simulink model "StampFly_KF400"  (R2026b)
settings: Solver=FixedStepDiscrete  StopTime=inf  FixedStep=Official.Step
PostLoadFcn:
  | run(fullfile(fileparts(get_param('StampFly_KF400','FileName')),'config','startup.m'));
InitFcn:
  | init_kf_flight;
undefined symbols (not defined in the file): AltitudeKF, Bottom, Discrete, Official, Time
libraries: slpidlib x7, simulink x4, ctrlSharedLib x1, mspfiltlib x1
(part 2 of 4)

== system StampFly_KF400/BottomRangeSensor400/BottomToF400 ==
  FinalMode : Inport
  BottomRangeBus : BusCreator  Inputs=2
  PreviousMode : UnitDelay  InitialCondition=uint8(0)  SampleTime=Official.Step
  RangeDiagnosticsBus : BusCreator  Inputs=3
  ToFReadyPoll400 : MATLABSystem  Description=下向きToF：Medium、33 ms。起動時のStartMeasurementは1回。dcnt>14とready割り込みでcore0へ読み出しを要求し、400 Hz側は待たず最新結果を取得。状態0の最遠対象[mm]、新着フラグ、測定状態を出力。前向きToFはXSHUT=LOWで無効。  Priority=3  System=official.BottomToF400  Sensor=Bottom (0x29)  I2CAddress=uint8( 41 )  SampleTime=Official.Step  DistanceMode=Auto (bottom Medium / front Long)  TimingBudget=20  PerformBringUp=on  TargetSelect=Auto (bottom Farthest / front Nearest)  SimulateUsing=Code generation
      mask Type: official.BottomToF400
  BottomRange : Outport
  RangeDiagnostics : Outport  Port=2
  wires:
  BottomRangeBus/1 -> BottomRange/1  "BottomRange"
  ToFReadyPoll400/5 -> RangeDiagnosticsBus/3  "Info"
  ToFReadyPoll400/4 -> RangeDiagnosticsBus/2  "Status"
  ToFReadyPoll400/3 -> RangeDiagnosticsBus/1  "FrontDistanceMm"
  FinalMode/1 -> PreviousMode/1
  ToFReadyPoll400/2 -> BottomRangeBus/2  "Fresh"
  PreviousMode/1 -> ToFReadyPoll400/1
  ToFReadyPoll400/1 -> BottomRangeBus/1  "DistanceMm"
  RangeDiagnosticsBus/1 -> RangeDiagnostics/1  "RangeDiagnostics"

== system StampFly_KF400/BottomRangeSensor400/JapaneseExplanation ==

== system StampFly_KF400/CommandPreparation400/FlightInputBus400 ==
  JoystickCommand : Inport
  BatteryVoltage : Inport  Port=2
  Dt : Inport  Port=3
  SensorStatus : Inport  Port=4
  CommandTapBus : BusCreator  Inputs=2
  ControlInputs : BusCreator  Inputs=7
  JoystickCommandFields : BusSelector  OutputSignals=Sticks,ArmButton,NewPacket,AHRSRequest
  SensorStatusFields : BusSelector  OutputSignals=Flags,Diagnostics
  SensorTapBus : BusCreator  Inputs=2
  FlightInputs : Outport
  CommandTap : Outport  Port=2
  SensorTap : Outport  Port=3
  wires:
  CommandTapBus/1 -> CommandTap/1  "CommandTap"
  SensorStatusFields/1 -> SensorTapBus/1, ControlInputs/7  "<Flags>"
  Dt/1 -> ControlInputs/6
  BatteryVoltage/1 -> ControlInputs/5
  JoystickCommandFields/4 -> CommandTapBus/2, ControlInputs/4  "<AHRSRequest>"
  ControlInputs/1 -> FlightInputs/1  "FlightInputs"
  JoystickCommand/1 -> JoystickCommandFields/1
  JoystickCommandFields/3 -> ControlInputs/3  "<NewPacket>"
  JoystickCommandFields/2 -> ControlInputs/2  "<ArmButton>"
  SensorStatus/1 -> SensorStatusFields/1
  JoystickCommandFields/1 -> CommandTapBus/1, ControlInputs/1  "<Sticks>"
  SensorStatusFields/2 -> SensorTapBus/2  "<Diagnostics>"
  SensorTapBus/1 -> SensorTap/1  "SensorTap"

== system StampFly_KF400/CommandPreparation400/JapaneseExplanation ==

== system StampFly_KF400/DataLogging50/JapaneseExplanation ==

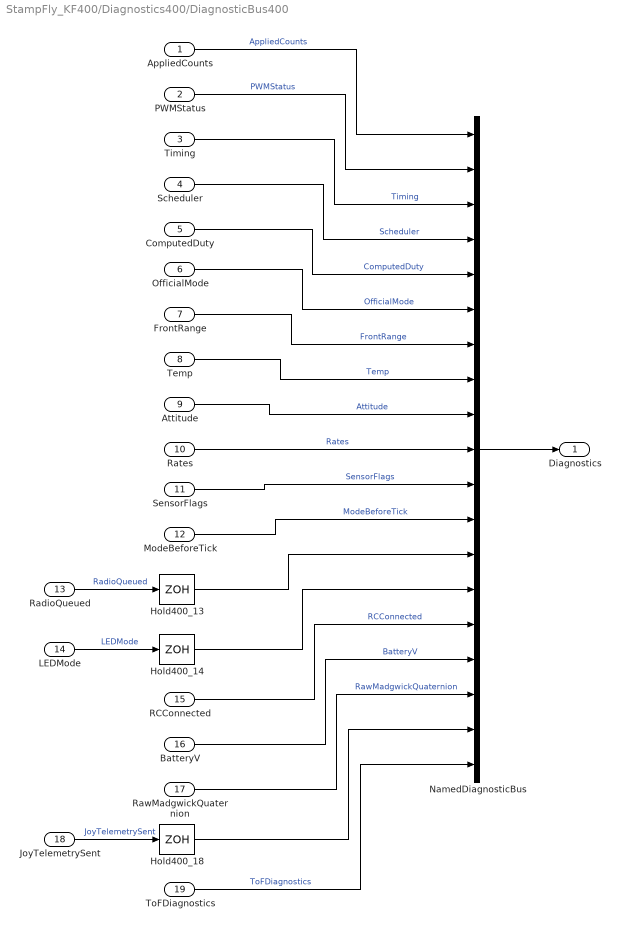
== system StampFly_KF400/Diagnostics400/DiagnosticBus400 ==
  AppliedCounts : Inport
  PWMStatus : Inport  Port=2
  Timing : Inport  Port=3
  Scheduler : Inport  Port=4
  ComputedDuty : Inport  Port=5
  OfficialMode : Inport  Port=6
  FrontRange : Inport  Port=7
  Temp : Inport  Port=8
  Attitude : Inport  Port=9
  Rates : Inport  Port=10
  SensorFlags : Inport  Port=11
  ModeBeforeTick : Inport  Port=12
  RadioQueued : Inport  Port=13
  LEDMode : Inport  Port=14
  RCConnected : Inport  Port=15
  BatteryV : Inport  Port=16
  RawMadgwickQuaternion : Inport  Port=17
  JoyTelemetrySent : Inport  Port=18
  ToFDiagnostics : Inport  Port=19
  Hold400_13 : ZeroOrderHold  SampleTime=.0025
  Hold400_14 : ZeroOrderHold  SampleTime=.0025
  Hold400_18 : ZeroOrderHold  SampleTime=.0025
  NamedDiagnosticBus : BusCreator  Inputs=19  OutDataTypeStr=Bus: OfficialDiagnosticBus  NonVirtualBus=on
  Diagnostics : Outport
  wires:
  RadioQueued/1 -> Hold400_13/1  "RadioQueued"
  ComputedDuty/1 -> NamedDiagnosticBus/5  "ComputedDuty"
  ModeBeforeTick/1 -> NamedDiagnosticBus/12  "ModeBeforeTick"
  Scheduler/1 -> NamedDiagnosticBus/4  "Scheduler"
  ToFDiagnostics/1 -> NamedDiagnosticBus/19  "ToFDiagnostics"
  SensorFlags/1 -> NamedDiagnosticBus/11  "SensorFlags"
  Timing/1 -> NamedDiagnosticBus/3  "Timing"
  Rates/1 -> NamedDiagnosticBus/10  "Rates"
  JoyTelemetrySent/1 -> Hold400_18/1  "JoyTelemetrySent"
  PWMStatus/1 -> NamedDiagnosticBus/2  "PWMStatus"
  RawMadgwickQuaternion/1 -> NamedDiagnosticBus/17  "RawMadgwickQuaternion"
  Attitude/1 -> NamedDiagnosticBus/9  "Attitude"
  AppliedCounts/1 -> NamedDiagnosticBus/1  "AppliedCounts"
  Hold400_14/1 -> NamedDiagnosticBus/14
  OfficialMode/1 -> NamedDiagnosticBus/6  "OfficialMode"
  LEDMode/1 -> Hold400_14/1  "LEDMode"
  RCConnected/1 -> NamedDiagnosticBus/15  "RCConnected"
  FrontRange/1 -> NamedDiagnosticBus/7  "FrontRange"
  BatteryV/1 -> NamedDiagnosticBus/16  "BatteryV"
  Temp/1 -> NamedDiagnosticBus/8  "Temp"
  Hold400_13/1 -> NamedDiagnosticBus/13
  Hold400_18/1 -> NamedDiagnosticBus/18
  NamedDiagnosticBus/1 -> Diagnostics/1

== system StampFly_KF400/EstimatorContext400/JapaneseExplanation ==

== system StampFly_KF400/FlightControl400/JapaneseExplanation ==

== system StampFly_KF400/FlightControl400/PreviousCycle400 ==
  ControlState : Inport
  SupervisorReset : Inport  Port=2
  AHRSResetMemory : UnitDelay  InitialCondition=false  SampleTime=Official.Step
  AltFlagMemory : UnitDelay  InitialCondition=uint8(0)  SampleTime=Official.Step
  AltFlagUInt8 : DataTypeConversion  OutDataTypeStr=uint8  SaturateOnIntegerOverflow=off  RndMeth=Floor
  ControlStateFields : BusSelector  OutputSignals=AltitudeEnabled,Mode
  EstimatorFeedbackBus : BusCreator  Inputs=4
  ModeMemory : UnitDelay  InitialCondition=uint8(0)  SampleTime=Official.Step
  ParkingResetMemory : UnitDelay  InitialCondition=false  SampleTime=Official.Step
  SupervisorResetFields : BusSelector  OutputSignals=AttitudeReset,ParkingReset
  EstimatorFeedback : Outport
  PreviousMode : Outport  Port=2
  AltitudeEnabled : Outport  Port=3
  wires:
  ControlStateFields/1 -> AltFlagUInt8/1  "<AltitudeEnabled>"
  SupervisorResetFields/1 -> AHRSResetMemory/1  "<AttitudeReset>"
  AltFlagMemory/1 -> EstimatorFeedbackBus/2  "AltitudeEnabled"
  ModeMemory/1 -> EstimatorFeedbackBus/1, PreviousMode/1  "PreviousMode"
  SupervisorReset/1 -> SupervisorResetFields/1
  ControlState/1 -> ControlStateFields/1
  ControlStateFields/2 -> ModeMemory/1  "<Mode>"
  SupervisorResetFields/2 -> ParkingResetMemory/1  "<ParkingReset>"
  ParkingResetMemory/1 -> EstimatorFeedbackBus/4  "ParkingReset"
  AltFlagUInt8/1 -> AltitudeEnabled/1, AltFlagMemory/1  "AltitudeEnabled"
  EstimatorFeedbackBus/1 -> EstimatorFeedback/1  "EstimatorFeedback"
  AHRSResetMemory/1 -> EstimatorFeedbackBus/3  "AttitudeReset"

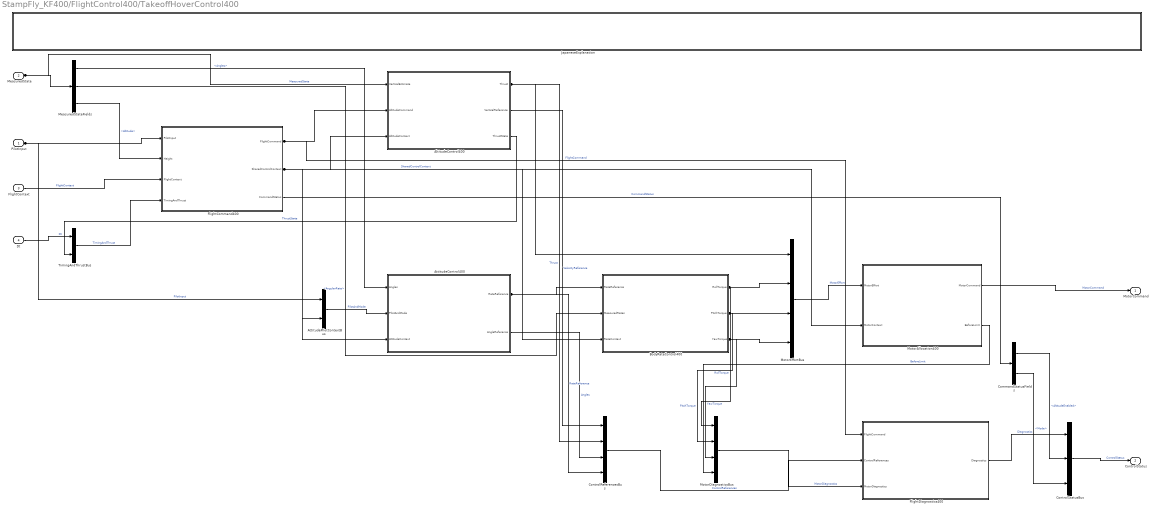
== system StampFly_KF400/FlightControl400/TakeoffHoverControl400 ==
  PilotInput : Inport
  MeasuredState : Inport  Port=2
  FlightContext : Inport  Port=3
  Dt : Inport  Port=4
  AltitudeControl400 : Subsystem  Description=高度PIDで鉛直速度指令を作り、鉛直速度PIDで共通推力を計算する。元の単精度PIDと遅延を保持。
      mask Display: disp('AltitudeControl400');port_label('input',1,'VerticalEstimate');port_label('input',2,'AltitudeCommand');port_label('input',3,'AltitudeContext');port_label('output',1,'Thrust');port_label('output',2,'VerticalReference');port_label('output',3,'ThrustState');
  AttitudeControl400 : Subsystem  Description=操縦入力を姿勢角・角速度指令に変換する。Stabilizeではロール・ピッチの姿勢角PIDを使う。
      mask Display: disp('AttitudeControl400');port_label('input',1,'Angles');port_label('input',2,'PilotAndMode');port_label('input',3,'AttitudeContext');port_label('output',1,'RateReference');port_label('output',2,'AngleReference');
  AttitudePilotContextBus : BusCreator  Inputs=2
  BodyRateControl400 : Subsystem  Description=指令角速度と実測ジャイロの差を3個のPIDで制御する。各軸のゲインは内部で個別に編集できる。
      mask Display: disp('BodyRateControl400');port_label('input',1,'RateReference');port_label('input',2,'MeasuredRates');port_label('input',3,'RateContext');port_label('output',1,'RollTorque');port_label('output',2,'PitchTorque');port_label('output',3,'YawTorque');
  CommandStatusFields : BusSelector  OutputSignals=AltitudeEnabled,Mode
  ControlReferencesBus : BusCreator  Inputs=4
  ControlStatusBus : BusCreator  Inputs=3
  FlightCommand400 : Subsystem  Description=飛行モードに応じた高度目標、推力の立ち上げ、PIDの実行・リセット条件を作る。内部のStateflowは既存の状態・遷移を保持。
      mask Display: disp('FlightCommand400');port_label('input',1,'PilotInput');port_label('input',2,'Height');port_label('input',3,'FlightContext');port_label('input',4,'TimingAndThrust');port_label('output',1,'FlightCommand');port_label('output',2,'SharedControlContext');port_label('output',3,'CommandStatus');
  FlightDiagnostics400 : Subsystem  Description=既存ロガーの制御診断ベクトルを元と同じ順序で作る。主制御の計算へは戻さない。
      mask Display: disp('FlightDiagnostics400');port_label('input',1,'FlightCommand');port_label('input',2,'ControlReferences');port_label('input',3,'MotorDiagnostics');port_label('output',1,'Diagnostics');
  JapaneseExplanation : Subsystem  Description=|
      | 離陸・ホバリング制御：400 Hz（2.5 ms）
      | 上段：高度・鉛直速度 → 共通推力。中段：姿勢角 → 角速度 → トルク → 4モーター。
      | 指令・条件は名前付きバスで直接配線。下段はロガー用の診断。各PIDは内部で個別に編集できます。
      mask Display: disp('離陸・ホバリング制御：400 Hz（2.5 ms）\n上段：高度・鉛直速度 → 共通推力。中段：姿勢角 → 角速度 → トルク → 4モーター。\n指令・条件は名前付きバスで直接配線。下段はロガー用の診断。各PIDは内部で個別に編集できます。')
  MeasuredStateFields : BusSelector  OutputSignals=Angles,AngularRate,Altitude
  MotorAllocation400 : Subsystem  Description=共通推力と3軸トルクをFR / FL / RR / RLに配分し、元の補正・制限・8 bit変換を行う。PWMのハードウェア書き込みは最上位の別ブロック。
      mask Display: disp('MotorAllocation400');port_label('input',1,'MotorEffort');port_label('input',2,'MotorContext');port_label('output',1,'MotorCommand');port_label('output',2,'BeforeLimit');
  MotorDiagnosticsBus : BusCreator  Inputs=4
  MotorEffortBus : BusCreator  Inputs=4
  TimingAndThrustBus : BusCreator  Inputs=2
  MotorCommand : Outport
  ControlStatus : Outport  Port=2
  wires:
  FlightContext/1 -> FlightCommand400/3(FlightContext)  "FlightContext"
  PilotInput/1 -> AttitudePilotContextBus/1, FlightCommand400/1(PilotInput)  "PilotInput"
  MeasuredState/1 -> AltitudeControl400/1(VerticalEstimate), MeasuredStateFields/1  "MeasuredState"
  FlightDiagnostics400/1(Diagnostics) -> ControlStatusBus/1  "Diagnostics"
  Dt/1 -> TimingAndThrustBus/1  "Dt"
  TimingAndThrustBus/1 -> FlightCommand400/4(TimingAndThrust)  "TimingAndThrust"
  AltitudeControl400/3(ThrustState) -> TimingAndThrustBus/2  "ThrustState"
  MeasuredStateFields/1 -> AttitudeControl400/1(Angles)  "<Angles>"
  MeasuredStateFields/2 -> BodyRateControl400/2(MeasuredRates)  "<AngularRate>"
  AltitudeControl400/2(VerticalReference) -> ControlReferencesBus/1  "VelocityReference"
  MeasuredStateFields/3 -> FlightCommand400/2(Height)  "<Altitude>"
  FlightCommand400/1(FlightCommand) -> AltitudeControl400/2(AltitudeCommand), FlightDiagnostics400/1(FlightCommand)  "FlightCommand"
  FlightCommand400/2(SharedControlContext) -> AttitudeControl400/3(AttitudeContext), MotorAllocation400/2(MotorContext), BodyRateControl400/3(RateContext), AltitudeControl400/3(AltitudeContext), AttitudePilotContextBus/2  "SharedControlContext"
  FlightCommand400/3(CommandStatus) -> CommandStatusFields/1  "CommandStatus"
  AltitudeControl400/1(Thrust) -> MotorEffortBus/1, ControlReferencesBus/2  "Thrust"
  AttitudePilotContextBus/1 -> AttitudeControl400/2(PilotAndMode)  "PilotAndMode"
  AttitudeControl400/1(RateReference) -> ControlReferencesBus/4, BodyRateControl400/1(RateReference)  "RateReference"
  AttitudeControl400/2(AngleReference) -> ControlReferencesBus/3  "Angles"
  ControlReferencesBus/1 -> FlightDiagnostics400/2(ControlReferences)  "ControlReferences"
  CommandStatusFields/2 -> ControlStatusBus/3  "<Mode>"
  BodyRateControl400/1(RollTorque) -> MotorDiagnosticsBus/1, MotorEffortBus/2  "RollTorque"
  MotorDiagnosticsBus/1 -> FlightDiagnostics400/3(MotorDiagnostics)  "MotorDiagnostics"
  BodyRateControl400/2(PitchTorque) -> MotorDiagnosticsBus/2, MotorEffortBus/3  "PitchTorque"
  BodyRateControl400/3(YawTorque) -> MotorDiagnosticsBus/3, MotorEffortBus/4  "YawTorque"
  MotorEffortBus/1 -> MotorAllocation400/1(MotorEffort)  "MotorEffort"
  MotorAllocation400/1(MotorCommand) -> MotorCommand/1  "MotorCommand"
  MotorAllocation400/2(BeforeLimit) -> MotorDiagnosticsBus/4  "BeforeLimit"
  CommandStatusFields/1 -> ControlStatusBus/2  "<AltitudeEnabled>"
  ControlStatusBus/1 -> ControlStatus/1  "ControlStatus"

== system StampFly_KF400/IMUSensor400/JapaneseExplanation ==

== system StampFly_KF400/JoystickCommand400/JoyStickInput400 ==
  BasicJoystick400 : MATLABSystem  Description=公式JoyStick受信：正しい送信元・宛先・CRCの25 byteだけが飛行通信を更新。ロガーからのパケットは飛行リンクを更新しない。  Priority=5  System=basic.Joystick400  SampleTime=.0025  Channel=uint8( 3 )  SimulateUsing=Code generation
      mask Type: basic.Joystick400
  JoystickCommandBus : BusCreator  Inputs=4  OutDataTypeStr=Bus: BasicLogPilotBus  NonVirtualBus=on
  PacketErrorDiagnostic : Terminator
  RadioDiagnosticsBus : BusCreator  Inputs=2
  RawLinkAgeUnused : Terminator
  JoystickCommand : Outport
  RadioDiagnostics : Outport  Port=2
  wires:
  BasicJoystick400/6 -> PacketErrorDiagnostic/1, RadioDiagnosticsBus/2  "PacketError"
  BasicJoystick400/1 -> JoystickCommandBus/1  "Sticks"
  BasicJoystick400/5 -> JoystickCommandBus/3  "NewPacket"
  BasicJoystick400/2 -> JoystickCommandBus/2  "ArmButton"
  BasicJoystick400/3 -> RawLinkAgeUnused/1, RadioDiagnosticsBus/1  "LinkAge"
  RadioDiagnosticsBus/1 -> RadioDiagnostics/1  "RadioDiagnostics"
  JoystickCommandBus/1 -> JoystickCommand/1  "JoystickCommand"
  BasicJoystick400/4 -> JoystickCommandBus/4  "AHRSRequest"

== system StampFly_KF400/JoystickFeedback40/JapaneseExplanation ==

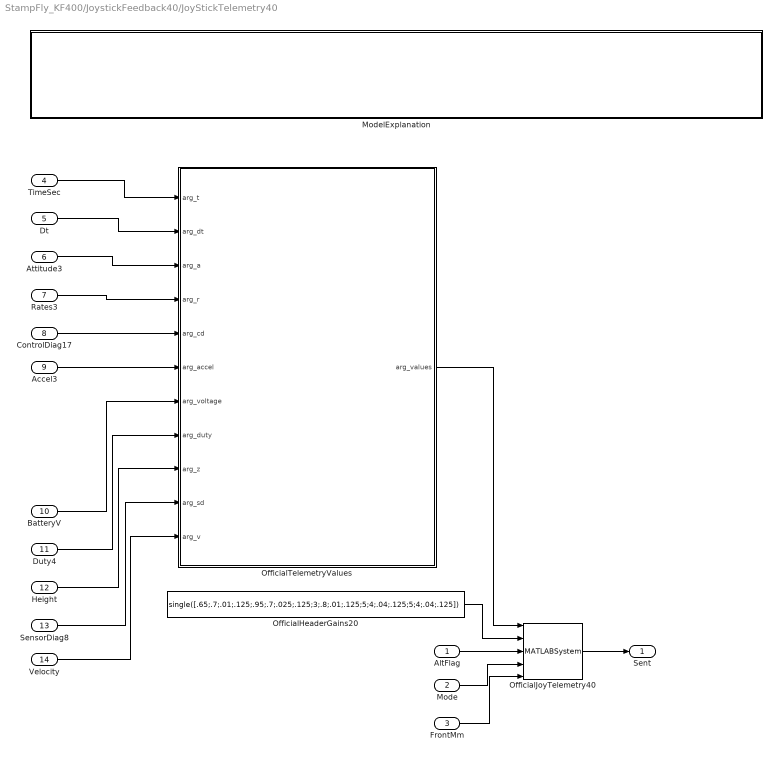
== system StampFly_KF400/JoystickFeedback40/JoyStickTelemetry40 ==
  AltFlag : Inport
  Mode : Inport  Port=2
  FrontMm : Inport  Port=3
  TimeSec : Inport  Port=4
  Dt : Inport  Port=5
  Attitude3 : Inport  Port=6
  Rates3 : Inport  Port=7
  ControlDiag17 : Inport  Port=8
  Accel3 : Inport  Port=9
  BatteryV : Inport  Port=10
  Duty4 : Inport  Port=11
  Height : Inport  Port=12
  SensorDiag8 : Inport  Port=13
  Velocity : Inport  Port=14
  ModelExplanation : Subsystem  Description=JoyStickへ公式テレメトリを40 Hzで返信。高度はSimulinkのKalman出力。前向きToFは無効（0）。
      mask Display: disp('説明\nJoyStickへ公式テレメトリを40 Hzで返信。高度はSimulinkのKalman出力。前向きToFは無効（0）。')
  OfficialHeaderGains20 : Constant  Value=single([.65;.7;.01;.125;.95;.7;.025;.125;3;.8;.01;.125;5;4;.04;.125;5;4;.04;.125])
  OfficialJoyTelemetry40 : MATLABSystem  Description=公式JoyStickへ40 Hzで高度・電圧・姿勢・モード等を返信します。  Priority=240  System=official.RadioTelemetryWrite40  SimulateUsing=Code generation
      mask Type: official.RadioTelemetryWrite40
  OfficialTelemetryValues : MATLAB Function  Description=計算処理。飛行状態遷移はStateflowで管理。  TreatAsAtomicUnit=on
  Sent : Outport
  wires:
  Attitude3/1 -> OfficialTelemetryValues/3(arg_a)
  TimeSec/1 -> OfficialTelemetryValues/1(arg_t)
  Dt/1 -> OfficialTelemetryValues/2(arg_dt)
  Duty4/1 -> OfficialTelemetryValues/8(arg_duty)
  Accel3/1 -> OfficialTelemetryValues/6(arg_accel)
  Rates3/1 -> OfficialTelemetryValues/4(arg_r)
  BatteryV/1 -> OfficialTelemetryValues/7(arg_voltage)
  ControlDiag17/1 -> OfficialTelemetryValues/5(arg_cd)
  Height/1 -> OfficialTelemetryValues/9(arg_z)
  SensorDiag8/1 -> OfficialTelemetryValues/10(arg_sd)
  Velocity/1 -> OfficialTelemetryValues/11(arg_v)
  OfficialTelemetryValues/1(arg_values) -> OfficialJoyTelemetry40/1
  OfficialHeaderGains20/1 -> OfficialJoyTelemetry40/2
  AltFlag/1 -> OfficialJoyTelemetry40/3
  Mode/1 -> OfficialJoyTelemetry40/4
  FrontMm/1 -> OfficialJoyTelemetry40/5
  OfficialJoyTelemetry40/1 -> Sent/1

== system StampFly_KF400/LEDAndBuzzer400/StatusOutputs400 ==
  Stick6 : Inport
  SensorFlags3 : Inport  Port=2
  ModeBeforeTick : Inport  Port=3
  AltFlag : Inport  Port=4
  PacketError : Inport  Port=5
  AHRSFlag : Inport  Port=6
  ControlMode : Selector  InputPortWidth=6  IndexOptions=Index vector (dialog)  Indices=5  OutputSizes=1
  LowVoltageCount : Selector  InputPortWidth=3  IndexOptions=Index vector (dialog)  Indices=3  OutputSizes=1
  ModelExplanation : Subsystem  Description=公式のモード・姿勢制御方式・高度制御・低電圧・通信エラーからLED色とブザー周波数を決定。ハードウェアはキュー送出のみ。
      mask Display: disp('説明\n公式のモード・姿勢制御方式・高度制御・低電圧・通信エラーからLED色とブザー周波数を決定。ハードウェアはキュー送出のみ。')
  StatusIndicators400 : MATLAB Function  Description=計算処理。飛行状態遷移はStateflowで管理。  TreatAsAtomicUnit=on
  StatusWrite400 : MATLABSystem  System=official.StatusWrite400  SimulateUsing=Code generation
      mask Type: official.StatusWrite400
  UserButton400 : MATLABSystem  System=official.UserButton400  SimulateUsing=Code generation
      mask Type: official.UserButton400
  wires:
  PacketError/1 -> StatusIndicators400/5(arg_rcError)
  LowVoltageCount/1 -> StatusIndicators400/4(arg_lowVoltage)
  ModeBeforeTick/1 -> StatusIndicators400/1(arg_mode)
  Stick6/1 -> ControlMode/1
  AHRSFlag/1 -> StatusIndicators400/6(arg_ahrsFlag)
  AltFlag/1 -> StatusIndicators400/3(arg_altFlag)
  SensorFlags3/1 -> LowVoltageCount/1
  ControlMode/1 -> StatusIndicators400/2(arg_controlMode)
  UserButton400/1 -> StatusIndicators400/7(arg_button)
  StatusIndicators400/1(arg_color1) -> StatusWrite400/1
  StatusIndicators400/2(arg_color2) -> StatusWrite400/2
  StatusIndicators400/3(arg_tone) -> StatusWrite400/3
  StatusIndicators400/4(arg_restart) -> StatusWrite400/4

== system StampFly_KF400/MagnetometerSensor400/JapaneseExplanation ==

== system StampFly_KF400/MotorWrite400/JapaneseExplanation ==

== system StampFly_KF400/MotorWrite400/MotorOutputs400 ==
  Counts4 : Inport
  ModelExplanation : Subsystem  Description=入力 Counts4 は FR / FL / RR / RL。LEDCキャリア150 kHz指定・8 bit、指令更新400 Hz。ベンチは定数Enable=falseとAllowMotorOutput=falseで実出力ゼロ。
      mask Display: disp('説明\n入力 Counts4 は FR / FL / RR / RL。LEDCキャリア150 kHz指定・8 bit、指令更新400 Hz。ベンチは定数Enable=falseとAllowMotorOutput=falseで実出力ゼロ。')
  MotorOutputEnabled : Constant  Value=true  SampleTime=Official.Step
  PWM150kHz8bit : MATLABSystem  Description=モーター書き込み：150 kHz指定、8 bit、FR/FL/RR/RL=GPIO42/5/41/10。実機ベンチではAllowMotorOutput=falseかつEnable=false、出力0です。  Priority=100  System=official.MotorPWM400  SampleTime=Official.Step  AllowMotorOutput=true  SimulateUsing=Code generation
      mask Type: official.MotorPWM400
  AppliedCounts4 : Outport
  PWMInfo4 : Outport  Port=2
  wires:
  PWM150kHz8bit/2 -> PWMInfo4/1
  Counts4/1 -> PWM150kHz8bit/1
  MotorOutputEnabled/1 -> PWM150kHz8bit/2
  PWM150kHz8bit/1 -> AppliedCounts4/1

== system StampFly_KF400/OpticalFlowDistance50/JapaneseExplanation ==

== system StampFly_KF400/OpticalFlowSensor400/JapaneseExplanation ==

== system StampFly_KF400/SensorCorrection400/IMUAxisConversion ==
  AccelMps2 : Inport
  GyroRps : Inport  Port=2
  AccelBodySigns : Product  Inputs=**
  AccelToG : Product  Inputs=*/
  BodyAxisSigns : Constant  Value=single([1;1;-1])
  GravityMps2 : Constant  Value=single(9.80665)
  GyroBodySigns : Product  Inputs=**
  JapaneseExplanation : Subsystem  Description=センサー座標から機体座標へ軸を入れ替え、符号と単位を変換します。姿勢推定・制御で同じ座標系を使うための処理です。
      mask Display: disp('センサー座標から機体座標へ軸を入れ替え、符号と単位を変換します。姿勢推定・制御で同じ座標系を使うための処理です。')
  SwapAccelXY : Selector  InputPortWidth=3  IndexOptions=Index vector (dialog)  Indices=[2 1 3]  OutputSizes=1
  SwapGyroXY : Selector  InputPortWidth=3  IndexOptions=Index vector (dialog)  Indices=[2 1 3]  OutputSizes=1
  BodyAccelG : Outport
  BodyGyroRps : Outport  Port=2
  wires:
  AccelMps2/1 -> SwapAccelXY/1
  AccelBodySigns/1 -> BodyAccelG/1
  GravityMps2/1 -> AccelToG/2
  SwapAccelXY/1 -> AccelToG/1
  AccelToG/1 -> AccelBodySigns/1
  GyroRps/1 -> SwapGyroXY/1
  SwapGyroXY/1 -> GyroBodySigns/1
  BodyAxisSigns/1 -> AccelBodySigns/2, GyroBodySigns/2
  GyroBodySigns/1 -> BodyGyroRps/1

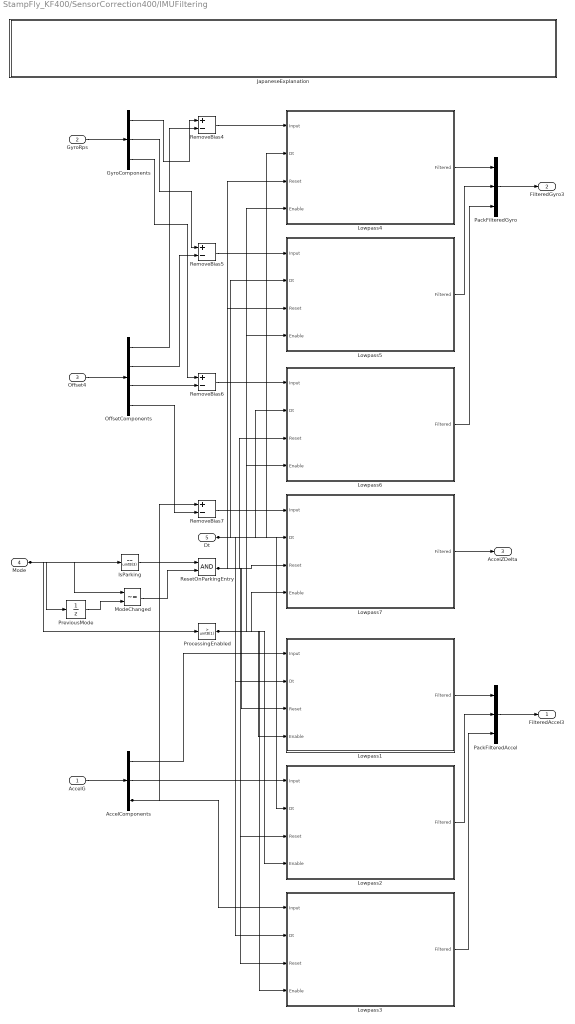
== system StampFly_KF400/SensorCorrection400/IMUFiltering ==
  AccelG : Inport
  GyroRps : Inport  Port=2
  Offset4 : Inport  Port=3
  Mode : Inport  Port=4
  Dt : Inport  Port=5
  AccelComponents : Demux  Outputs=3
  GyroComponents : Demux  Outputs=3
  IsParking : simulink/Logic and Bit Operations/Compare To Constant  relop===  const=uint8(3)  OutDataTypeStr=boolean
  JapaneseExplanation : Subsystem  Description=|
      | IMUフィルター（400 Hz）
      | 加速度・角速度のバイアス補正と低域フィルター。鉛直加速度の変化も出力。
      | 各軸のSum / Gain / Unit Delayを編集して、元の演算順を確認できます。
      mask Display: disp('IMUフィルター（400 Hz）\n加速度・角速度のバイアス補正と低域フィルター。鉛直加速度の変化も出力。\n各軸のSum / Gain / Unit Delayを編集して、元の演算順を確認できます。')
  Lowpass1 : Subsystem
  Lowpass2 : Subsystem
  Lowpass3 : Subsystem
  Lowpass4 : Subsystem
  Lowpass5 : Subsystem
  Lowpass6 : Subsystem
  Lowpass7 : Subsystem
  ModeChanged : RelationalOperator  Operator=~=  OutDataTypeStr=boolean  RndMeth=Simplest  InputSameDT=off
  OffsetComponents : Demux
  PackFilteredAccel : Mux  Inputs=3
  PackFilteredGyro : Mux  Inputs=3
  PreviousMode : UnitDelay  InitialCondition=uint8(0)  SampleTime=.0025
  ProcessingEnabled : simulink/Logic and Bit Operations/Compare To Constant  relop=>  const=uint8(1)  OutDataTypeStr=boolean
  RemoveBias{4..7} (4 alike) : Sum  Inputs=+-
  ResetOnParkingEntry : Logic  IconShape=distinctive  AllPortsSameDT=off  OutDataTypeStr=boolean
  FilteredAccel3 : Outport
  FilteredGyro3 : Outport  Port=2
  AccelZDelta : Outport  Port=3
  wires:
  Mode/1 -> IsParking/1, ModeChanged/1, ProcessingEnabled/1, PreviousMode/1
  PreviousMode/1 -> ModeChanged/2
  GyroComponents/3 -> RemoveBias6/1
  GyroRps/1 -> GyroComponents/1
  Lowpass6/1(Filtered) -> PackFilteredGyro/3
  Offset4/1 -> OffsetComponents/1
  OffsetComponents/3 -> RemoveBias6/2
  GyroComponents/1 -> RemoveBias4/1
  AccelG/1 -> AccelComponents/1
  GyroComponents/2 -> RemoveBias5/1
  OffsetComponents/1 -> RemoveBias4/2
  OffsetComponents/2 -> RemoveBias5/2
  OffsetComponents/4 -> RemoveBias7/2
  ModeChanged/1 -> ResetOnParkingEntry/2
  IsParking/1 -> ResetOnParkingEntry/1
  AccelComponents/1 -> Lowpass1/1(Input)
  AccelComponents/2 -> Lowpass2/1(Input)
  AccelComponents/3 -> Lowpass3/1(Input), RemoveBias7/1
  Lowpass3/1(Filtered) -> PackFilteredAccel/3
  RemoveBias4/1 -> Lowpass4/1(Input)
  RemoveBias5/1 -> Lowpass5/1(Input)
  RemoveBias6/1 -> Lowpass6/1(Input)
  RemoveBias7/1 -> Lowpass7/1(Input)
  Dt/1 -> Lowpass5/2(Dt), Lowpass7/2(Dt), Lowpass3/2(Dt), Lowpass6/2(Dt), Lowpass1/2(Dt), Lowpass4/2(Dt), Lowpass2/2(Dt)
  ResetOnParkingEntry/1 -> Lowpass2/3(Reset), Lowpass7/3(Reset), Lowpass1/3(Reset), Lowpass4/3(Reset), Lowpass5/3(Reset), Lowpass6/3(Reset), Lowpass3/3(Reset)
  ProcessingEnabled/1 -> Lowpass2/4(Enable), Lowpass1/4(Enable), Lowpass4/4(Enable), Lowpass7/4(Enable), Lowpass3/4(Enable), Lowpass6/4(Enable), Lowpass5/4(Enable)
  Lowpass4/1(Filtered) -> PackFilteredGyro/1
  Lowpass5/1(Filtered) -> PackFilteredGyro/2
  Lowpass7/1(Filtered) -> AccelZDelta/1
  Lowpass1/1(Filtered) -> PackFilteredAccel/1
  Lowpass2/1(Filtered) -> PackFilteredAccel/2
  PackFilteredGyro/1 -> FilteredGyro3/1
  PackFilteredAccel/1 -> FilteredAccel3/1

== system StampFly_KF400/SensorCorrection400/JapaneseExplanation ==

== system StampFly_KF400/SensorCorrection400/VerticalAcceleration ==
  AccelZDelta : Inport
  Mode : Inport  Port=2
  Dt : Inport  Port=3
  IsParking : simulink/Logic and Bit Operations/Compare To Constant  relop===  const=uint8(3)  OutDataTypeStr=boolean
  JapaneseExplanation : Subsystem  Description=加速度Zの変化を公式と同じ低域フィルターで処理し、高度Kalmanへ渡す鉛直加速度を作ります。
      mask Display: disp('加速度Zの変化を公式と同じ低域フィルターで処理し、高度Kalmanへ渡す鉛直加速度を作ります。')
  ModeChanged : RelationalOperator  Operator=~=  OutDataTypeStr=boolean  RndMeth=Simplest  InputSameDT=off
  PreviousMode : UnitDelay  InitialCondition=uint8(0)  SampleTime=.0025
  ProcessingEnabled : simulink/Logic and Bit Operations/Compare To Constant  relop=>  const=uint8(1)  OutDataTypeStr=boolean
  ResetOnParkingEntry : Logic  IconShape=distinctive  AllPortsSameDT=off  OutDataTypeStr=boolean
  UpwardSign : Gain  Gain=single(-1)
  VerticalLowpass : Subsystem
  VerticalAccel : Outport
  wires:
  ProcessingEnabled/1 -> VerticalLowpass/4(Enable)
  Mode/1 -> ModeChanged/1, ProcessingEnabled/1, IsParking/1, PreviousMode/1
  PreviousMode/1 -> ModeChanged/2
  IsParking/1 -> ResetOnParkingEntry/1
  AccelZDelta/1 -> UpwardSign/1
  Dt/1 -> VerticalLowpass/2(Dt)
  ModeChanged/1 -> ResetOnParkingEntry/2
  UpwardSign/1 -> VerticalLowpass/1(Input)
  ResetOnParkingEntry/1 -> VerticalLowpass/3(Reset)
  VerticalLowpass/1(Filtered) -> VerticalAccel/1

== system StampFly_KF400/AttitudeAltitudeEstimation400/AltitudeKalman/FilterStep ==
  AltitudeM : Inport
  AccelerationG : Inport  Port=2
  Dt : Inport  Port=3
  A : Inport  Port=4
  B : Inport  Port=5
  C : Inport  Port=6
  Q : Inport  Port=7
  Reset : Inport  Port=8
  ProcessParameters : Inport  Port=9
  Enable : EnablePort
  AdvanceCorrectedState : MATLAB Function  TreatAsAtomicUnit=on
  InitialCovariance : Constant  Value=AltitudeKF.InitialCovariance  VectorParams1D=off
  KalmanFilter : ctrlSharedLib/Kalman Filter  TimeDomain=Discrete-Time  UseCurrentEstimator=on  ModelSource=Input port  ModelSourceVariable=ss(0.95,1,1,0,1)  A=0.95  B=1  C=1  D=0  NumberOfStates=3  NumberOfInputs=1  NumberOfOutputs=1  Ts=AltitudeKF.SampleTime  InitialEstimateSource=Input port  X0=0  P0=10  UseK=off  UseGH=off  G=1  TimeInvariantG=on  H=0  TimeInvariantH=on  NumberOfProcessNoiseInputs=1  Q=0.05  TimeInvariantQ=off  R=AltitudeKF.MeasurementVariance  TimeInvariantR=on  N=zeros(3,1,'single')  TimeInvariantN=on  AddInputPort=on  AddEnablePort=off  ExternalReset=Level hold  OutputEstimatedY=off  OutputP=off
  RetainedPrivateState : UnitDelay  InitialCondition=AltitudeKF.InitialState  SampleTime=-1
  ZeroFeedthrough : Constant  Value=single(0)
  StateVector : Outport  InitialOutput=AltitudeKF.InitialState
  wires:
  AdvanceCorrectedState/1(state) -> RetainedPrivateState/1, StateVector/1
  ProcessParameters/1 -> AdvanceCorrectedState/4(processParameters)
  Dt/1 -> AdvanceCorrectedState/3(dt)
  KalmanFilter/1 -> AdvanceCorrectedState/1(xhat)
  Reset/1 -> KalmanFilter/5
  InitialCovariance/1 -> KalmanFilter/4
  RetainedPrivateState/1 -> KalmanFilter/3
  Q/1 -> KalmanFilter/10
  ZeroFeedthrough/1 -> KalmanFilter/9
  C/1 -> KalmanFilter/8
  B/1 -> KalmanFilter/7
  A/1 -> KalmanFilter/6
  AltitudeM/1 -> KalmanFilter/2
  AccelerationG/1 -> KalmanFilter/1, AdvanceCorrectedState/2(az)

== system StampFly_KF400/AttitudeAltitudeEstimation400/IMUAttitude400/FusionState ==
  Accel : Inport  PortDimensions=[1 3]
  Gyro : Inport  Port=2  PortDimensions=[1 3]
  Reset : Inport  Port=3
  Enable : EnablePort
  UpdateWhenReady : Subsystem
  Orientation : Outport  PortDimensions=[1 4]  InitialOutput=single([1 0 0 0])
  AngularVelocity : Outport  Port=2  PortDimensions=[1 3]  InitialOutput=single([0 0 0])
  wires:
  UpdateWhenReady/2(AngularVelocity) -> AngularVelocity/1
  UpdateWhenReady/1(Orientation) -> Orientation/1
  Reset/1 -> UpdateWhenReady/Reset
  Gyro/1 -> UpdateWhenReady/2(Gyro)
  Accel/1 -> UpdateWhenReady/1(Accel)

== system StampFly_KF400/FlightControl400/TakeoffHoverControl400/AltitudeControl400 ==
  VerticalEstimate : Inport
  AltitudeCommand : Inport  Port=2
  AltitudeContext : Inport  Port=3
  AltitudeCommandFields : BusSelector  OutputSignals=HeightReference,BaseThrust,AltitudeEnabled,ManualAltitude
  AltitudeContextFields : BusSelector  OutputSignals=ThrustRequest,ControlContext.VelocityEnabled,ControlContext.AltitudeEnabled,ControlContext.Reset,FlightContext.Branch,Mode,Dt,PreviousError
  AltitudeError : Sum  Inputs=+-
  AltitudePID : Subsystem  Description=専用PIDの飛行比較版：AltitudePID。Enable停止中は出力・状態を保持。Resetは実行中に反映。PreviousError入力は未使用。元PIDとは厳密等価ではない。
  HeldThrustMemory : UnitDelay  InitialCondition=single(0)  SampleTime=Official.Step
  SelectVerticalReference : MATLAB Function  Description=|  TreatAsAtomicUnit=on
      | 自動高度 / 着陸 -0.15 m/s
      | 計算処理。飛行状態遷移はStateflowで管理。
  ThrustCorrectionLimits : MATLAB Function  Description=|  TreatAsAtomicUnit=on
      | 基準推力 / フィルター / 上下限
      | 計算処理。飛行状態遷移はStateflowで管理。
  ThrustFilterMemory : UnitDelay  InitialCondition=single(0)  SampleTime=Official.Step
  ThrustStateBus : BusCreator  Inputs=2
  VerticalEstimateFields : BusSelector  OutputSignals=Altitude,Velocity
  VerticalSpeedError : Sum  Inputs=+-
  VerticalSpeedPID : Subsystem  Description=専用PIDの飛行比較版：VerticalSpeedPID。Enable停止中は出力・状態を保持。Resetは実行中に反映。PreviousError入力は未使用。元PIDとは厳密等価ではない。
  Thrust : Outport
  VerticalReference : Outport  Port=2
  ThrustState : Outport  Port=3
  wires:
  AltitudeError/1 -> AltitudePID/1(Error)
  AltitudeCommandFields/2 -> ThrustCorrectionLimits/3(arg_arg_base)  "<BaseThrust>"
  AltitudeContextFields/8 -> AltitudePID/5(PreviousError), VerticalSpeedPID/5(PreviousError)  "<PreviousError>"
  AltitudeContext/1 -> AltitudeContextFields/1
  AltitudeContextFields/6 -> SelectVerticalReference/2(arg_mode)  "<Mode>"
  AltitudeCommand/1 -> AltitudeCommandFields/1
  AltitudeContextFields/4 -> VerticalSpeedPID/4(Reset), AltitudePID/4(Reset)  "<Reset>"
  VerticalEstimate/1 -> VerticalEstimateFields/1
  VerticalEstimateFields/1 -> AltitudeError/2  "<Altitude>"
  VerticalEstimateFields/2 -> VerticalSpeedError/2  "<Velocity>"
  AltitudeCommandFields/3 -> SelectVerticalReference/3(arg_auto), ThrustCorrectionLimits/4(arg_arg_auto)  "<AltitudeEnabled>"
  AltitudeCommandFields/1 -> AltitudeError/1  "<HeightReference>"
  AltitudeCommandFields/4 -> ThrustCorrectionLimits/5(arg_arg_manual)  "<ManualAltitude>"
  AltitudeContextFields/1 -> ThrustCorrectionLimits/1(arg_arg_command)  "<ThrustRequest>"
  AltitudeContextFields/2 -> VerticalSpeedPID/3(Enable), ThrustCorrectionLimits/6(arg_arg_velEnable)  "<VelocityEnabled>"
  AltitudePID/1(Output) -> SelectVerticalReference/1(arg_zRef), VerticalReference/1  "VelocityReference"
  AltitudeContextFields/3 -> AltitudePID/3(Enable)  "<AltitudeEnabled>"
  AltitudeContextFields/5 -> ThrustCorrectionLimits/7(arg_branch)  "<Branch>"
  AltitudeContextFields/7 -> ThrustCorrectionLimits/8(arg_arg_dt), AltitudePID/2(Dt), VerticalSpeedPID/2(Dt)  "<Dt>"
  SelectVerticalReference/1(arg_vRef) -> VerticalSpeedError/1
  VerticalSpeedError/1 -> VerticalSpeedPID/1(Error)
  VerticalSpeedPID/1(Output) -> ThrustCorrectionLimits/2(arg_arg_correction)
  ThrustFilterMemory/1 -> ThrustStateBus/1, ThrustCorrectionLimits/9(arg_arg_oldFilter)  "FilteredThrust"
  ThrustCorrectionLimits/1(arg_arg_thrust) -> Thrust/1  "Thrust"
  ThrustCorrectionLimits/2(arg_arg_filter) -> ThrustFilterMemory/1
  ThrustCorrectionLimits/3(arg_arg_last) -> HeldThrustMemory/1
  HeldThrustMemory/1 -> ThrustCorrectionLimits/10(arg_arg_lastThrust), ThrustStateBus/2  "HeldThrust"
  ThrustStateBus/1 -> ThrustState/1  "ThrustState"

== system StampFly_KF400/FlightControl400/TakeoffHoverControl400/AttitudeControl400 ==
  Angles : Inport
  PilotAndMode : Inport  Port=2
  AttitudeContext : Inport  Port=3
  AngleTargets : Demux  Outputs=2
  AttitudeContextFields : BusSelector  OutputSignals=ControlContext.Run,ControlContext.Reset,ControlContext.AngleEnabled,Dt
  EstimatedAngles : Demux  Outputs=3
  LastRateReference : UnitDelay  InitialCondition=zeros(3,1,'single')  SampleTime=Official.Step
  PilotAndModeFields : BusSelector  OutputSignals=PilotInput.Sticks,SharedControlContext.FlightContext.Branch,SharedControlContext.ControlMode
  PitchAngleError : Sum  Inputs=+-
  PitchAnglePID : Subsystem  Description=専用PIDの飛行比較版：PitchAnglePID。Enable停止中は出力・状態を保持。Resetは実行中に反映。PreviousError入力は未使用。元PIDとは厳密等価ではない。
  ResetPreviousAngles : Demux  Outputs=2
  RollAngleError : Sum  Inputs=+-
  RollAnglePID : Subsystem  Description=専用PIDの飛行比較版：RollAnglePID。Enable停止中は出力・状態を保持。Resetは実行中に反映。PreviousError入力は未使用。元PIDとは厳密等価ではない。
  SelectRateReference : MATLAB Function  Description=|  TreatAsAtomicUnit=on
      | 姿勢 PID / Sport
      | 計算処理。飛行状態遷移はStateflowで管理。
  StickToAngleRate : MATLAB Function  Description=|  TreatAsAtomicUnit=on
      | Stabilize / Sport
      | 計算処理。飛行状態遷移はStateflowで管理。
  UnusedYaw : Terminator
  RateReference : Outport
  AngleReference : Outport  Port=2
  wires:
  AttitudeContextFields/2 -> PitchAnglePID/4(Reset), RollAnglePID/4(Reset), StickToAngleRate/4(arg_arg_reset)  "<Reset>"
  PilotAndModeFields/2 -> StickToAngleRate/2(arg_branch)  "<Branch>"
  AttitudeContext/1 -> AttitudeContextFields/1
  EstimatedAngles/2 -> PitchAngleError/2
  PilotAndMode/1 -> PilotAndModeFields/1
  AttitudeContextFields/3 -> RollAnglePID/3(Enable), PitchAnglePID/3(Enable), SelectRateReference/4(angleEnable)  "<AngleEnabled>"
  PilotAndModeFields/3 -> StickToAngleRate/6(arg_arg_controlMode)  "<ControlMode>"
  AttitudeContextFields/1 -> StickToAngleRate/3(arg_arg_run)  "<Run>"
  StickToAngleRate/1(arg_arg_angle) -> AngleReference/1, AngleTargets/1  "AngleReference"
  PilotAndModeFields/1 -> StickToAngleRate/1(arg_arg_stick)  "<Sticks>"
  AttitudeContextFields/4 -> RollAnglePID/2(Dt), PitchAnglePID/2(Dt)  "<Dt>"
  StickToAngleRate/2(arg_arg_directRate) -> SelectRateReference/1(direct)
  AngleTargets/2 -> PitchAngleError/1
  StickToAngleRate/3(arg_arg_resetError) -> ResetPreviousAngles/1
  Angles/1 -> EstimatedAngles/1
  AngleTargets/1 -> RollAngleError/1
  EstimatedAngles/1 -> RollAngleError/2
  EstimatedAngles/3 -> UnusedYaw/1
  RollAngleError/1 -> RollAnglePID/1(Error)
  PitchAngleError/1 -> PitchAnglePID/1(Error)
  ResetPreviousAngles/1 -> RollAnglePID/5(PreviousError)
  ResetPreviousAngles/2 -> PitchAnglePID/5(PreviousError)
  RollAnglePID/1(Output) -> SelectRateReference/2(rollPID)
  LastRateReference/1 -> StickToAngleRate/5(arg_arg_lastRate)
  PitchAnglePID/1(Output) -> SelectRateReference/3(pitchPID)
  SelectRateReference/1(rate) -> LastRateReference/1, RateReference/1  "RateReference"

== system StampFly_KF400/FlightControl400/TakeoffHoverControl400/BodyRateControl400 ==
  RateReference : Inport
  MeasuredRates : Inport  Port=2
  RateContext : Inport  Port=3
  EstimatedRates : Demux  Outputs=3
  PitchRateError : Sum  Inputs=+-
  PitchRatePID : Subsystem  Description=専用PIDの飛行比較版：PitchRatePID。Enable停止中は出力・状態を保持。Resetは実行中に反映。PreviousError入力は未使用。元PIDとは厳密等価ではない。
  RateContextFields : BusSelector  OutputSignals=ControlContext.Run,ControlContext.Reset,Dt,PreviousError
  RollRateError : Sum  Inputs=+-
  RollRatePID : Subsystem  Description=専用PIDの飛行比較版：RollRatePID。Enable停止中は出力・状態を保持。Resetは実行中に反映。PreviousError入力は未使用。元PIDとは厳密等価ではない。
  TargetRates : Demux  Outputs=3
  YawRateError : Sum  Inputs=+-
  YawRatePID : Subsystem  Description=専用PIDの飛行比較版：YawRatePID。Enable停止中は出力・状態を保持。Resetは実行中に反映。PreviousError入力は未使用。元PIDとは厳密等価ではない。
  RollTorque : Outport
  PitchTorque : Outport  Port=2
  YawTorque : Outport  Port=3
  wires:
  EstimatedRates/2 -> PitchRateError/2
  RateReference/1 -> TargetRates/1
  MeasuredRates/1 -> EstimatedRates/1
  TargetRates/1 -> RollRateError/1
  TargetRates/2 -> PitchRateError/1
  TargetRates/3 -> YawRateError/1
  EstimatedRates/1 -> RollRateError/2
  EstimatedRates/3 -> YawRateError/2
  RateContext/1 -> RateContextFields/1
  RollRateError/1 -> RollRatePID/1(Error)
  PitchRateError/1 -> PitchRatePID/1(Error)
  YawRateError/1 -> YawRatePID/1(Error)
  RateContextFields/1 -> RollRatePID/3(Enable), PitchRatePID/3(Enable), YawRatePID/3(Enable)  "<Run>"
  RateContextFields/2 -> RollRatePID/4(Reset), PitchRatePID/4(Reset), YawRatePID/4(Reset)  "<Reset>"
  RateContextFields/3 -> RollRatePID/2(Dt), PitchRatePID/2(Dt), YawRatePID/2(Dt)  "<Dt>"
  RateContextFields/4 -> RollRatePID/5(PreviousError), PitchRatePID/5(PreviousError), YawRatePID/5(PreviousError)  "<PreviousError>"
  RollRatePID/1(Output) -> RollTorque/1  "RollTorque"
  PitchRatePID/1(Output) -> PitchTorque/1  "PitchTorque"
  YawRatePID/1(Output) -> YawTorque/1  "YawTorque"

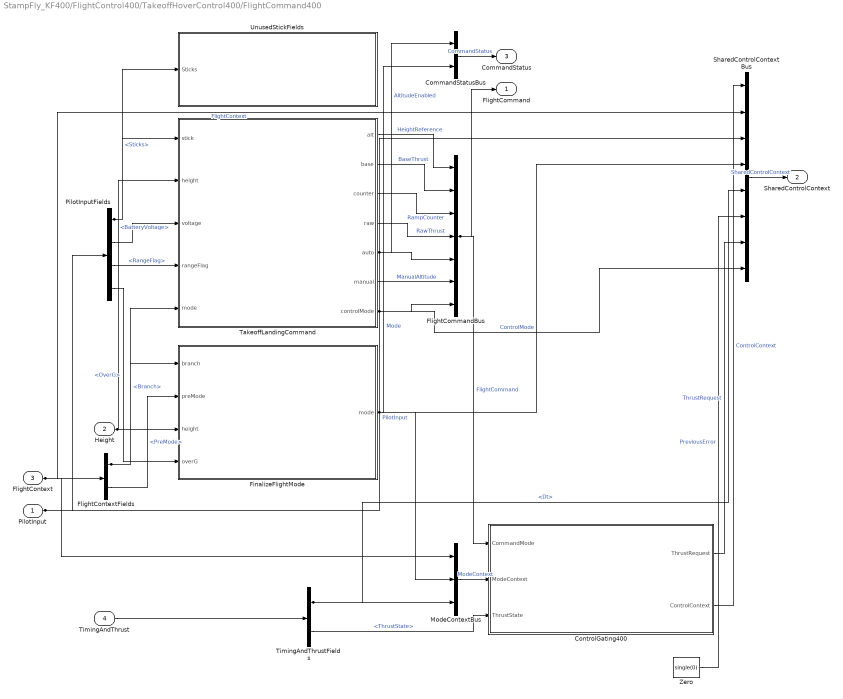
== system StampFly_KF400/FlightControl400/TakeoffHoverControl400/FlightCommand400 ==
  PilotInput : Inport
  Height : Inport  Port=2
  FlightContext : Inport  Port=3
  TimingAndThrust : Inport  Port=4
  CommandStatusBus : BusCreator  Inputs=2
  ControlGating400 : Subsystem  Description=元の判定と演算を保持し、各PIDの実行・保持・リセット条件を名前付きバスで出力する。
      mask Display: disp('ControlGating400');port_label('input',1,'CommandMode');port_label('input',2,'ModeContext');port_label('input',3,'ThrustState');port_label('output',1,'ThrustRequest');port_label('output',2,'ControlContext');
  FinalizeFlightMode : Stateflow chart  Description=元の状態遷移を保持し、着陸完了・異常時の最終モードを確定する。  TreatAsAtomicUnit=on
  FlightCommandBus : BusCreator  Inputs=7
  FlightContextFields : BusSelector  OutputSignals=Branch,PreMode
  ModeContextBus : BusCreator  Inputs=3
  PilotInputFields : BusSelector  OutputSignals=Sticks,BatteryVoltage,RangeFlag,OverG
  SharedControlContextBus : BusCreator  Inputs=8
  TakeoffLandingCommand : Stateflow chart  Description=元の離陸・着陸の状態遷移を保持。自動高度の初期目標0.5 mと推力立ち上げを生成する。  TreatAsAtomicUnit=on
  TimingAndThrustFields : BusSelector  OutputSignals=Dt,ThrustState
  UnusedStickFields : Subsystem  Description=元のブロックと接続を維持した表示用のサブシステムです。
  Zero : Constant  Value=single(0)
  FlightCommand : Outport
  SharedControlContext : Outport  Port=2
  CommandStatus : Outport  Port=3
  wires:
  CommandStatusBus/1 -> CommandStatus/1  "CommandStatus"
  PilotInputFields/2 -> TakeoffLandingCommand/3(voltage)  "<BatteryVoltage>"
  TakeoffLandingCommand/2(base) -> FlightCommandBus/2  "BaseThrust"
  PilotInput/1 -> SharedControlContextBus/3, PilotInputFields/1  "PilotInput"
  TakeoffLandingCommand/6(manual) -> FlightCommandBus/6  "ManualAltitude"
  FlightContext/1 -> ModeContextBus/1, SharedControlContextBus/2, FlightContextFields/1  "FlightContext"
  PilotInputFields/1 -> UnusedStickFields/1(Sticks), TakeoffLandingCommand/1(stick)  "<Sticks>"
  PilotInputFields/3 -> TakeoffLandingCommand/4(rangeFlag)  "<RangeFlag>"
  TimingAndThrustFields/2 -> ControlGating400/3(ThrustState)  "<ThrustState>"
  TakeoffLandingCommand/4(raw) -> FlightCommandBus/4  "RawThrust"
  FlightContextFields/1 -> FinalizeFlightMode/1(branch), TakeoffLandingCommand/5(mode)  "<Branch>"
  PilotInputFields/4 -> FinalizeFlightMode/4(overG)  "<OverG>"
  Height/1 -> TakeoffLandingCommand/2(height), FinalizeFlightMode/3(height)
  TakeoffLandingCommand/5(auto) -> FlightCommandBus/5, CommandStatusBus/1  "AltitudeEnabled"
  FlightContextFields/2 -> FinalizeFlightMode/2(preMode)  "<PreMode>"
  TimingAndThrust/1 -> TimingAndThrustFields/1
  TakeoffLandingCommand/1(alt) -> FlightCommandBus/1  "HeightReference"
  TimingAndThrustFields/1 -> SharedControlContextBus/5, ModeContextBus/3  "<Dt>"
  TakeoffLandingCommand/3(counter) -> FlightCommandBus/3  "RampCounter"
  TakeoffLandingCommand/7(controlMode) -> SharedControlContextBus/8, FlightCommandBus/7  "ControlMode"
  FinalizeFlightMode/1(mode) -> CommandStatusBus/2, SharedControlContextBus/4, ModeContextBus/2  "Mode"
  FlightCommandBus/1 -> ControlGating400/1(CommandMode), FlightCommand/1  "FlightCommand"
  ModeContextBus/1 -> ControlGating400/2(ModeContext)  "ModeContext"
  ControlGating400/1(ThrustRequest) -> SharedControlContextBus/7  "ThrustRequest"
  ControlGating400/2(ControlContext) -> SharedControlContextBus/1  "ControlContext"
  Zero/1 -> SharedControlContextBus/6  "PreviousError"
  SharedControlContextBus/1 -> SharedControlContext/1  "SharedControlContext"

== system StampFly_KF400/FlightControl400/TakeoffHoverControl400/FlightDiagnostics400 ==
  FlightCommand : Inport
  ControlReferences : Inport  Port=2
  MotorDiagnostics : Inport  Port=3
  ControlDiagnosticPack : MATLAB Function  Description=|  TreatAsAtomicUnit=on
      | 目標・補正量・配分前出力
      | 計算処理。飛行状態遷移はStateflowで管理。
  ControlReferencesFields : BusSelector  OutputSignals=VelocityReference,Thrust,Angles,RateReference
  FlightCommandFields : BusSelector  OutputSignals=HeightReference,BaseThrust,RampCounter
  MotorDiagnosticsFields : BusSelector  OutputSignals=RollTorque,PitchTorque,YawTorque,BeforeLimit
  Diagnostics : Outport
  wires:
  MotorDiagnostics/1 -> MotorDiagnosticsFields/1
  FlightCommand/1 -> FlightCommandFields/1
  ControlReferences/1 -> ControlReferencesFields/1
  FlightCommandFields/1 -> ControlDiagnosticPack/1(alt)  "<HeightReference>"
  FlightCommandFields/2 -> ControlDiagnosticPack/2(base)  "<BaseThrust>"
  ControlReferencesFields/1 -> ControlDiagnosticPack/4(zRef)  "<VelocityReference>"
  FlightCommandFields/3 -> ControlDiagnosticPack/3(counter)  "<RampCounter>"
  ControlReferencesFields/2 -> ControlDiagnosticPack/5(thrust)  "<Thrust>"
  ControlReferencesFields/3 -> ControlDiagnosticPack/6(angle)  "<Angles>"
  ControlReferencesFields/4 -> ControlDiagnosticPack/7(rate)  "<RateReference>"
  MotorDiagnosticsFields/1 -> ControlDiagnosticPack/8(rollTorque)  "<RollTorque>"
  MotorDiagnosticsFields/2 -> ControlDiagnosticPack/9(pitchTorque)  "<PitchTorque>"
  MotorDiagnosticsFields/3 -> ControlDiagnosticPack/10(yawTorque)  "<YawTorque>"
  MotorDiagnosticsFields/4 -> ControlDiagnosticPack/11(before)  "<BeforeLimit>"
  ControlDiagnosticPack/1(diag) -> Diagnostics/1  "Diagnostics"

== system StampFly_KF400/FlightControl400/TakeoffHoverControl400/JapaneseExplanation ==

== system StampFly_KF400/FlightControl400/TakeoffHoverControl400/MotorAllocation400 ==
  MotorEffort : Inport
  MotorContext : Inport  Port=2
  MotorCommandBus : BusCreator  Inputs=2
  MotorContextFields : BusSelector  OutputSignals=ControlContext.Run,ControlContext.Reset,PilotInput.OverG,FlightContext.Branch,Dt
  MotorEffortFields : BusSelector  OutputSignals=Thrust,RollTorque,PitchTorque,YawTorque
  MotorMixerFilter8bit : Subsystem  Description=4ch / Duty 0〜0.95 / 8 bit
      mask Display: disp('MotorMixerFilter8bit');port_label('input',1,'Thrust');port_label('input',2,'RollTorque');port_label('input',3,'PitchTorque');port_label('input',4,'YawTorque');port_label('input',5,'Run');port_label('input',6,'Reset');port_label('input',7,'OverG');port_label('input',8,'Mode');port_label('input',9,'Dt');port_label('output',1,'Duty4');port_label('output',2,'Counts4');port_label('output',3,'BeforeLimit4');
  MotorCommand : Outport
  BeforeLimit : Outport  Port=2
  wires:
  MotorEffortFields/1 -> MotorMixerFilter8bit/1(Thrust)  "<Thrust>"
  MotorMixerFilter8bit/3(BeforeLimit4) -> BeforeLimit/1  "BeforeLimit"
  MotorEffort/1 -> MotorEffortFields/1
  MotorContextFields/2 -> MotorMixerFilter8bit/6(Reset)  "<Reset>"
  MotorEffortFields/3 -> MotorMixerFilter8bit/3(PitchTorque)  "<PitchTorque>"
  MotorContext/1 -> MotorContextFields/1
  MotorContextFields/1 -> MotorMixerFilter8bit/5(Run)  "<Run>"
  MotorEffortFields/2 -> MotorMixerFilter8bit/2(RollTorque)  "<RollTorque>"
  MotorEffortFields/4 -> MotorMixerFilter8bit/4(YawTorque)  "<YawTorque>"
  MotorContextFields/3 -> MotorMixerFilter8bit/7(OverG)  "<OverG>"
  MotorContextFields/4 -> MotorMixerFilter8bit/8(Mode)  "<Branch>"
  MotorContextFields/5 -> MotorMixerFilter8bit/9(Dt)  "<Dt>"
  MotorMixerFilter8bit/1(Duty4) -> MotorCommandBus/1  "Duty"
  MotorMixerFilter8bit/2(Counts4) -> MotorCommandBus/2  "Counts"
  MotorCommandBus/1 -> MotorCommand/1  "MotorCommand"

== system StampFly_KF400/JoystickFeedback40/JoyStickTelemetry40/ModelExplanation ==

== system StampFly_KF400/LEDAndBuzzer400/StatusOutputs400/ModelExplanation ==

== system StampFly_KF400/MotorWrite400/MotorOutputs400/ModelExplanation ==

== system StampFly_KF400/SensorCorrection400/IMUAxisConversion/JapaneseExplanation ==

== system StampFly_KF400/SensorCorrection400/IMUFiltering/JapaneseExplanation ==

== system StampFly_KF400/SensorCorrection400/IMUFiltering/Lowpass1 ==
  Input : Inport
  Dt : Inport  Port=2
  Reset : Inport  Port=3
  Enable : Inport  Port=4
  Denominator : Sum
  InputTerm : Product  Inputs=*/
  InputTimesDt : Product  Inputs=**
  PreviousFiltered : UnitDelay  InitialCondition=single(0)  SampleTime=.0025
  PreviousTerm : Product  Inputs=*/
  PreviousTimesT : Product  Inputs=**
  ResetPrevious : Switch  Criteria=u2 ~= 0  SaturateOnIntegerOverflow=off  InputSameDT=off
  TimeConstantS : Constant  Value=single(0.0030000000000000001)
  UpdateOrHold : Switch  Criteria=u2 ~= 0  SaturateOnIntegerOverflow=off  InputSameDT=off
  UpdatedFiltered : Sum
  ZeroOnReset : Constant  Value=single(0)
  Filtered : Outport
  wires:
  Input/1 -> InputTimesDt/1
  Denominator/1 -> PreviousTerm/2, InputTerm/2
  InputTimesDt/1 -> InputTerm/1
  Dt/1 -> Denominator/2, InputTimesDt/2
  TimeConstantS/1 -> PreviousTimesT/2, Denominator/1
  Enable/1 -> UpdateOrHold/2
  InputTerm/1 -> UpdatedFiltered/2
  UpdatedFiltered/1 -> UpdateOrHold/1
  UpdateOrHold/1 -> PreviousFiltered/1, Filtered/1
  ZeroOnReset/1 -> ResetPrevious/1
  Reset/1 -> ResetPrevious/2
  PreviousFiltered/1 -> ResetPrevious/3
  ResetPrevious/1 -> UpdateOrHold/3, PreviousTimesT/1
  PreviousTimesT/1 -> PreviousTerm/1
  PreviousTerm/1 -> UpdatedFiltered/1

== system StampFly_KF400/SensorCorrection400/IMUFiltering/Lowpass2 ==
  Input : Inport
  Dt : Inport  Port=2
  Reset : Inport  Port=3
  Enable : Inport  Port=4
  Denominator : Sum
  InputTerm : Product  Inputs=*/
  InputTimesDt : Product  Inputs=**
  PreviousFiltered : UnitDelay  InitialCondition=single(0)  SampleTime=.0025
  PreviousTerm : Product  Inputs=*/
  PreviousTimesT : Product  Inputs=**
  ResetPrevious : Switch  Criteria=u2 ~= 0  SaturateOnIntegerOverflow=off  InputSameDT=off
  TimeConstantS : Constant  Value=single(0.0030000000000000001)
  UpdateOrHold : Switch  Criteria=u2 ~= 0  SaturateOnIntegerOverflow=off  InputSameDT=off
  UpdatedFiltered : Sum
  ZeroOnReset : Constant  Value=single(0)
  Filtered : Outport
  wires:
  Input/1 -> InputTimesDt/1
  Denominator/1 -> PreviousTerm/2, InputTerm/2
  InputTimesDt/1 -> InputTerm/1
  Dt/1 -> Denominator/2, InputTimesDt/2
  TimeConstantS/1 -> Denominator/1, PreviousTimesT/2
  Enable/1 -> UpdateOrHold/2
  InputTerm/1 -> UpdatedFiltered/2
  UpdatedFiltered/1 -> UpdateOrHold/1
  UpdateOrHold/1 -> PreviousFiltered/1, Filtered/1
  ZeroOnReset/1 -> ResetPrevious/1
  Reset/1 -> ResetPrevious/2
  PreviousFiltered/1 -> ResetPrevious/3
  ResetPrevious/1 -> UpdateOrHold/3, PreviousTimesT/1
  PreviousTimesT/1 -> PreviousTerm/1
  PreviousTerm/1 -> UpdatedFiltered/1

== system StampFly_KF400/SensorCorrection400/IMUFiltering/Lowpass3 ==
  Input : Inport
  Dt : Inport  Port=2
  Reset : Inport  Port=3
  Enable : Inport  Port=4
  Denominator : Sum
  InputTerm : Product  Inputs=*/
  InputTimesDt : Product  Inputs=**
  PreviousFiltered : UnitDelay  InitialCondition=single(0)  SampleTime=.0025
  PreviousTerm : Product  Inputs=*/
  PreviousTimesT : Product  Inputs=**
  ResetPrevious : Switch  Criteria=u2 ~= 0  SaturateOnIntegerOverflow=off  InputSameDT=off
  TimeConstantS : Constant  Value=single(0.0030000000000000001)
  UpdateOrHold : Switch  Criteria=u2 ~= 0  SaturateOnIntegerOverflow=off  InputSameDT=off
  UpdatedFiltered : Sum
  ZeroOnReset : Constant  Value=single(0)
  Filtered : Outport
  wires:
  Input/1 -> InputTimesDt/1
  Denominator/1 -> PreviousTerm/2, InputTerm/2
  InputTimesDt/1 -> InputTerm/1
  Dt/1 -> Denominator/2, InputTimesDt/2
  TimeConstantS/1 -> PreviousTimesT/2, Denominator/1
  Enable/1 -> UpdateOrHold/2
  InputTerm/1 -> UpdatedFiltered/2
  UpdatedFiltered/1 -> UpdateOrHold/1
  UpdateOrHold/1 -> PreviousFiltered/1, Filtered/1
  ZeroOnReset/1 -> ResetPrevious/1
  Reset/1 -> ResetPrevious/2
  PreviousFiltered/1 -> ResetPrevious/3
  ResetPrevious/1 -> PreviousTimesT/1, UpdateOrHold/3
  PreviousTimesT/1 -> PreviousTerm/1
  PreviousTerm/1 -> UpdatedFiltered/1

== system StampFly_KF400/SensorCorrection400/IMUFiltering/Lowpass4 ==
  Input : Inport
  Dt : Inport  Port=2
  Reset : Inport  Port=3
  Enable : Inport  Port=4
  Denominator : Sum
  InputTerm : Product  Inputs=*/
  InputTimesDt : Product  Inputs=**
  PreviousFiltered : UnitDelay  InitialCondition=single(0)  SampleTime=.0025
  PreviousTerm : Product  Inputs=*/
  PreviousTimesT : Product  Inputs=**
  ResetPrevious : Switch  Criteria=u2 ~= 0  SaturateOnIntegerOverflow=off  InputSameDT=off
  TimeConstantS : Constant  Value=single(0.0030000000000000001)
  UpdateOrHold : Switch  Criteria=u2 ~= 0  SaturateOnIntegerOverflow=off  InputSameDT=off
  UpdatedFiltered : Sum
  ZeroOnReset : Constant  Value=single(0)
  Filtered : Outport
  wires:
  Input/1 -> InputTimesDt/1
  Denominator/1 -> PreviousTerm/2, InputTerm/2
  InputTimesDt/1 -> InputTerm/1
  Dt/1 -> Denominator/2, InputTimesDt/2
  TimeConstantS/1 -> PreviousTimesT/2, Denominator/1
  Enable/1 -> UpdateOrHold/2
  InputTerm/1 -> UpdatedFiltered/2
  UpdatedFiltered/1 -> UpdateOrHold/1
  UpdateOrHold/1 -> PreviousFiltered/1, Filtered/1
  ZeroOnReset/1 -> ResetPrevious/1
  Reset/1 -> ResetPrevious/2
  PreviousFiltered/1 -> ResetPrevious/3
  ResetPrevious/1 -> PreviousTimesT/1, UpdateOrHold/3
  PreviousTimesT/1 -> PreviousTerm/1
  PreviousTerm/1 -> UpdatedFiltered/1

== system StampFly_KF400/SensorCorrection400/IMUFiltering/Lowpass5 ==
  Input : Inport
  Dt : Inport  Port=2
  Reset : Inport  Port=3
  Enable : Inport  Port=4
  Denominator : Sum
  InputTerm : Product  Inputs=*/
  InputTimesDt : Product  Inputs=**
  PreviousFiltered : UnitDelay  InitialCondition=single(0)  SampleTime=.0025
  PreviousTerm : Product  Inputs=*/
  PreviousTimesT : Product  Inputs=**
  ResetPrevious : Switch  Criteria=u2 ~= 0  SaturateOnIntegerOverflow=off  InputSameDT=off
  TimeConstantS : Constant  Value=single(0.0030000000000000001)
  UpdateOrHold : Switch  Criteria=u2 ~= 0  SaturateOnIntegerOverflow=off  InputSameDT=off
  UpdatedFiltered : Sum
  ZeroOnReset : Constant  Value=single(0)
  Filtered : Outport
  wires:
  Input/1 -> InputTimesDt/1
  Denominator/1 -> PreviousTerm/2, InputTerm/2
  InputTimesDt/1 -> InputTerm/1
  Dt/1 -> Denominator/2, InputTimesDt/2
  TimeConstantS/1 -> PreviousTimesT/2, Denominator/1
  Enable/1 -> UpdateOrHold/2
  InputTerm/1 -> UpdatedFiltered/2
  UpdatedFiltered/1 -> UpdateOrHold/1
  UpdateOrHold/1 -> PreviousFiltered/1, Filtered/1
  ZeroOnReset/1 -> ResetPrevious/1
  Reset/1 -> ResetPrevious/2
  PreviousFiltered/1 -> ResetPrevious/3
  ResetPrevious/1 -> UpdateOrHold/3, PreviousTimesT/1
  PreviousTimesT/1 -> PreviousTerm/1
  PreviousTerm/1 -> UpdatedFiltered/1
